simulink model "ts_b02f_log"  (R2024b)
settings: Solver=FixedStepDiscrete  StartTime=0.0  StopTime=10  FixedStep=Ts  RelTol=1e-4
PreLoadFcn:
  | Ts=50e-6;
undefined symbols (not defined in the file): D1, Delta, DiscIntNeverNeededParam
libraries: simulink x22, spsSecondOrderFilterLib x14, spsThreePhaseVIMeasurementLib x7, spsabctodq0Lib x6, spsThreePhaseSeriesRLCLoadLib x5, spsPowerPLLDrivenPositiveSequenceLib x4, spsStairGeneratorLib x4, spsThreePhaseTransformerTwoWindingsLib x3, spsDCVoltageSourceLib x3, spsThreePhaseSeriesRLCBranchLib x3, spsPWMGeneratorPulseAveragingLib x3, spsTwoLevelConverterLib x3
(part 3 of 3)

== system ts_b02f_log/Inverter 2 300 kW/Control System/Current Regulator/PI regulator with anti-windup D ==
  note: Anti-windup mechanism: Method of conditionnal integration
      |
      | The integration is suspended if saturation occurs and the
      | control error is of the same sign as the control signal.
      |
      | [1] L.Rundqwist, "Anti-Reset Windup for PID Controllers," Ph.D. Thesis TRFT-1033,
      | Departement of Automatic Control, Lund Institute of Technology, Lund, Sweeden, 1991.
  Error : Inport  SampleTime=Ts
  Compare To Zero : simulink/Logic and Bit Operations/Compare To Zero  relop=>  OutDataTypeStr=uint8  ZeroCross=off
  Compare To Zero1 : simulink/Logic and Bit Operations/Compare To Zero  relop=<  OutDataTypeStr=uint8  ZeroCross=off
  Constant : Constant  Value=0
  Constant1 : Constant  Value=UpperLimit
  Constant3 : Constant  Value=LowerLimit
  Discrete-Time Integrator : DiscreteIntegrator  IntegratorMethod=Integration: Trapezoidal  InitialCondition=Init  SampleTime=Ts  LimitOutput=on  UpperSaturationLimit=UpperLimit  LowerSaturationLimit=LowerLimit  ShowStatePort=on  ICPrevOutput=DiscIntNeverNeededParam  ICPrevScaledInput=DiscIntNeverNeededParam
  Kp4 : Gain  Gain=Kp  SaturateOnIntegerOverflow=on  SampleTime=Ts  OutDataTypeStr=Inherit: Same as input  ParamDataTypeStr=Inherit: Same as input
  Kp5 : Gain  Gain=Ki  SaturateOnIntegerOverflow=on  SampleTime=Ts  OutDataTypeStr=Inherit: Same as input  ParamDataTypeStr=Inherit: Same as input
  Logical Operator : Logic  AllPortsSameDT=off  OutDataTypeStr=boolean
  Logical Operator1 : Logic  AllPortsSameDT=off  OutDataTypeStr=boolean
  Logical Operator2 : Logic  Operator=OR  AllPortsSameDT=off  OutDataTypeStr=boolean
  Relational Operator : RelationalOperator  OutDataTypeStr=boolean  InputSameDT=off
  Relational Operator1 : RelationalOperator  Operator=<=  OutDataTypeStr=boolean  InputSameDT=off
  Saturation2 : Saturate  UpperLimit=UpperLimit  LowerLimit=LowerLimit  SampleTime=Ts
  Sum1 : Sum  InputSameDT=on  SaturateOnIntegerOverflow=on  SampleTime=Ts  OutDataTypeStr=Inherit: Same as first input
  Sum6 : Sum  InputSameDT=on  SaturateOnIntegerOverflow=on  SampleTime=Ts  OutDataTypeStr=Inherit: Same as first input
  Switch : Switch  Criteria=u2 > Threshold  SaturateOnIntegerOverflow=off  InputSameDT=off
  Zero-Order Hold : ZeroOrderHold  SampleTime=Ts
  Out : Outport  SampleTime=Ts  InitialOutput=0  VectorParamsAs1DForOutWhenUnconnected=off
  wires:
  Constant/1 -> Switch/1
  Zero-Order Hold/1 -> Sum1/2, Sum6/1
  Discrete-Time Integrator/State -> Sum1/1
  Sum1/1 -> Relational Operator1/1, Relational Operator/1
  Logical Operator2/1 -> Switch/2
  Relational Operator/1 -> Logical Operator/1  "UpperLimit_is_Reached"
  Relational Operator1/1 -> Logical Operator1/1  "LowerLimit_Is_Reached"
  Constant1/1 -> Relational Operator/2
  Constant3/1 -> Relational Operator1/2
  Compare To Zero/1 -> Logical Operator/2  "Error_is_positive"
  Logical Operator/1 -> Logical Operator2/1
  Logical Operator1/1 -> Logical Operator2/2
  Compare To Zero1/1 -> Logical Operator1/2  "Error_is_negative"
  Error/1 -> Compare To Zero1/1, Compare To Zero/1, Kp4/1, Kp5/1
  Sum6/1 -> Saturation2/1
  Kp4/1 -> Zero-Order Hold/1
  Discrete-Time Integrator/1 -> Sum6/2
  Saturation2/1 -> Out/1
  Switch/1 -> Discrete-Time Integrator/1
  Kp5/1 -> Switch/3

== system ts_b02f_log/Inverter 2 300 kW/Control System/Voltage Regulators/PI regulator with anti-windup 1 ==
  note: Anti-windup mechanism: Method of conditionnal integration
      |
      | The integration is suspended if saturation occurs and the
      | control error is of the same sign as the control signal.
      |
      | [1] L.Rundqwist, "Anti-Reset Windup for PID Controllers," Ph.D. Thesis TRFT-1033,
      | Departement of Automatic Control, Lund Institute of Technology, Lund, Sweeden, 1991.
  Error : Inport  SampleTime=Ts
  Reset : Inport  Port=2  SampleTime=Ts
  Compare To Zero : simulink/Logic and Bit Operations/Compare To Zero  relop=>  OutDataTypeStr=uint8  ZeroCross=off
  Compare To Zero1 : simulink/Logic and Bit Operations/Compare To Zero  relop=<  OutDataTypeStr=uint8  ZeroCross=off
  Constant : Constant  Value=0
  Constant1 : Constant  Value=UpperLimit
  Constant3 : Constant  Value=LowerLimit
  Discrete-Time Integrator : DiscreteIntegrator  IntegratorMethod=Integration: Trapezoidal  ExternalReset=level  InitialCondition=Init  SampleTime=Ts  LimitOutput=on  UpperSaturationLimit=UpperLimit  LowerSaturationLimit=LowerLimit  ShowStatePort=on  ICPrevOutput=DiscIntNeverNeededParam  ICPrevScaledInput=DiscIntNeverNeededParam
  Kp4 : Gain  Gain=Kp  SaturateOnIntegerOverflow=on  SampleTime=Ts  OutDataTypeStr=Inherit: Same as input  ParamDataTypeStr=Inherit: Same as input
  Kp5 : Gain  Gain=Ki  SaturateOnIntegerOverflow=on  SampleTime=Ts  OutDataTypeStr=Inherit: Same as input  ParamDataTypeStr=Inherit: Same as input
  Logical Operator : Logic  AllPortsSameDT=off  OutDataTypeStr=boolean
  Logical Operator1 : Logic  AllPortsSameDT=off  OutDataTypeStr=boolean
  Logical Operator2 : Logic  Operator=OR  AllPortsSameDT=off  OutDataTypeStr=boolean
  Relational Operator : RelationalOperator  OutDataTypeStr=boolean  InputSameDT=off
  Relational Operator1 : RelationalOperator  Operator=<=  OutDataTypeStr=boolean  InputSameDT=off
  Saturation2 : Saturate  UpperLimit=UpperLimit  LowerLimit=LowerLimit  SampleTime=Ts
  Sum1 : Sum  InputSameDT=on  SaturateOnIntegerOverflow=on  SampleTime=Ts  OutDataTypeStr=Inherit: Same as first input
  Sum6 : Sum  InputSameDT=on  SaturateOnIntegerOverflow=on  SampleTime=Ts  OutDataTypeStr=Inherit: Same as first input
  Switch : Switch  Criteria=u2 > Threshold  SaturateOnIntegerOverflow=off  InputSameDT=off
  Zero-Order Hold : ZeroOrderHold  SampleTime=Ts
  Out : Outport  SampleTime=Ts  InitialOutput=0  VectorParamsAs1DForOutWhenUnconnected=off
  wires:
  Kp5/1 -> Switch/3
  Switch/1 -> Discrete-Time Integrator/1
  Saturation2/1 -> Out/1
  Discrete-Time Integrator/1 -> Sum6/2
  Kp4/1 -> Zero-Order Hold/1
  Sum6/1 -> Saturation2/1
  Error/1 -> Kp5/1, Kp4/1, Compare To Zero/1, Compare To Zero1/1
  Compare To Zero1/1 -> Logical Operator1/2  "Error_is_negative"
  Logical Operator1/1 -> Logical Operator2/2
  Logical Operator/1 -> Logical Operator2/1
  Compare To Zero/1 -> Logical Operator/2  "Error_is_positive"
  Constant3/1 -> Relational Operator1/2
  Constant1/1 -> Relational Operator/2
  Relational Operator1/1 -> Logical Operator1/1  "LowerLimit_Is_Reached"
  Relational Operator/1 -> Logical Operator/1  "UpperLimit_is_Reached"
  Logical Operator2/1 -> Switch/2
  Sum1/1 -> Relational Operator/1, Relational Operator1/1
  Discrete-Time Integrator/State -> Sum1/1
  Zero-Order Hold/1 -> Sum6/1, Sum1/2
  Constant/1 -> Switch/1
  Reset/1 -> Discrete-Time Integrator/2

== system ts_b02f_log/Inverter 2 300 kW/Control System/Voltage Regulators/PI regulator with anti-windup 2 ==
  note: Anti-windup mechanism: Method of conditionnal integration
      |
      | The integration is suspended if saturation occurs and the
      | control error is of the same sign as the control signal.
      |
      | [1] L.Rundqwist, "Anti-Reset Windup for PID Controllers," Ph.D. Thesis TRFT-1033,
      | Departement of Automatic Control, Lund Institute of Technology, Lund, Sweeden, 1991.
  Error : Inport  SampleTime=Ts
  Reset : Inport  Port=2  SampleTime=Ts
  Compare To Zero : simulink/Logic and Bit Operations/Compare To Zero  relop=>  OutDataTypeStr=uint8  ZeroCross=off
  Compare To Zero1 : simulink/Logic and Bit Operations/Compare To Zero  relop=<  OutDataTypeStr=uint8  ZeroCross=off
  Constant : Constant  Value=0
  Constant1 : Constant  Value=UpperLimit
  Constant3 : Constant  Value=LowerLimit
  Discrete-Time Integrator : DiscreteIntegrator  IntegratorMethod=Integration: Trapezoidal  ExternalReset=level  InitialCondition=Init  SampleTime=Ts  LimitOutput=on  UpperSaturationLimit=UpperLimit  LowerSaturationLimit=LowerLimit  ShowStatePort=on  ICPrevOutput=DiscIntNeverNeededParam  ICPrevScaledInput=DiscIntNeverNeededParam
  Kp4 : Gain  Gain=Kp  SaturateOnIntegerOverflow=on  SampleTime=Ts  OutDataTypeStr=Inherit: Same as input  ParamDataTypeStr=Inherit: Same as input
  Kp5 : Gain  Gain=Ki  SaturateOnIntegerOverflow=on  SampleTime=Ts  OutDataTypeStr=Inherit: Same as input  ParamDataTypeStr=Inherit: Same as input
  Logical Operator : Logic  AllPortsSameDT=off  OutDataTypeStr=boolean
  Logical Operator1 : Logic  AllPortsSameDT=off  OutDataTypeStr=boolean
  Logical Operator2 : Logic  Operator=OR  AllPortsSameDT=off  OutDataTypeStr=boolean
  Relational Operator : RelationalOperator  OutDataTypeStr=boolean  InputSameDT=off
  Relational Operator1 : RelationalOperator  Operator=<=  OutDataTypeStr=boolean  InputSameDT=off
  Saturation2 : Saturate  UpperLimit=UpperLimit  LowerLimit=LowerLimit  SampleTime=Ts
  Sum1 : Sum  InputSameDT=on  SaturateOnIntegerOverflow=on  SampleTime=Ts  OutDataTypeStr=Inherit: Same as first input
  Sum6 : Sum  InputSameDT=on  SaturateOnIntegerOverflow=on  SampleTime=Ts  OutDataTypeStr=Inherit: Same as first input
  Switch : Switch  Criteria=u2 > Threshold  SaturateOnIntegerOverflow=off  InputSameDT=off
  Zero-Order Hold : ZeroOrderHold  SampleTime=Ts
  Out : Outport  SampleTime=Ts  InitialOutput=0  VectorParamsAs1DForOutWhenUnconnected=off
  wires:
  Kp5/1 -> Switch/3
  Switch/1 -> Discrete-Time Integrator/1
  Saturation2/1 -> Out/1
  Discrete-Time Integrator/1 -> Sum6/2
  Kp4/1 -> Zero-Order Hold/1
  Sum6/1 -> Saturation2/1
  Error/1 -> Kp5/1, Kp4/1, Compare To Zero/1, Compare To Zero1/1
  Compare To Zero1/1 -> Logical Operator1/2  "Error_is_negative"
  Logical Operator1/1 -> Logical Operator2/2
  Logical Operator/1 -> Logical Operator2/1
  Compare To Zero/1 -> Logical Operator/2  "Error_is_positive"
  Constant3/1 -> Relational Operator1/2
  Constant1/1 -> Relational Operator/2
  Relational Operator1/1 -> Logical Operator1/1  "LowerLimit_Is_Reached"
  Relational Operator/1 -> Logical Operator/1  "UpperLimit_is_Reached"
  Logical Operator2/1 -> Switch/2
  Sum1/1 -> Relational Operator/1, Relational Operator1/1
  Discrete-Time Integrator/State -> Sum1/1
  Zero-Order Hold/1 -> Sum6/1, Sum1/2
  Constant/1 -> Switch/1
  Reset/1 -> Discrete-Time Integrator/2

== system ts_b02f_log/Inverter 3 200 kW/Control System/Current Regulator/PI regulator with anti-windup D ==
  note: Anti-windup mechanism: Method of conditionnal integration
      |
      | The integration is suspended if saturation occurs and the
      | control error is of the same sign as the control signal.
      |
      | [1] L.Rundqwist, "Anti-Reset Windup for PID Controllers," Ph.D. Thesis TRFT-1033,
      | Departement of Automatic Control, Lund Institute of Technology, Lund, Sweeden, 1991.
  Error : Inport  SampleTime=Ts
  Compare To Zero : simulink/Logic and Bit Operations/Compare To Zero  relop=>  OutDataTypeStr=uint8  ZeroCross=off
  Compare To Zero1 : simulink/Logic and Bit Operations/Compare To Zero  relop=<  OutDataTypeStr=uint8  ZeroCross=off
  Constant : Constant  Value=0
  Constant1 : Constant  Value=UpperLimit
  Constant3 : Constant  Value=LowerLimit
  Discrete-Time Integrator : DiscreteIntegrator  IntegratorMethod=Integration: Trapezoidal  InitialCondition=Init  SampleTime=Ts  LimitOutput=on  UpperSaturationLimit=UpperLimit  LowerSaturationLimit=LowerLimit  ShowStatePort=on  ICPrevOutput=DiscIntNeverNeededParam  ICPrevScaledInput=DiscIntNeverNeededParam
  Kp4 : Gain  Gain=Kp  SaturateOnIntegerOverflow=on  SampleTime=Ts  OutDataTypeStr=Inherit: Same as input  ParamDataTypeStr=Inherit: Same as input
  Kp5 : Gain  Gain=Ki  SaturateOnIntegerOverflow=on  SampleTime=Ts  OutDataTypeStr=Inherit: Same as input  ParamDataTypeStr=Inherit: Same as input
  Logical Operator : Logic  AllPortsSameDT=off  OutDataTypeStr=boolean
  Logical Operator1 : Logic  AllPortsSameDT=off  OutDataTypeStr=boolean
  Logical Operator2 : Logic  Operator=OR  AllPortsSameDT=off  OutDataTypeStr=boolean
  Relational Operator : RelationalOperator  OutDataTypeStr=boolean  InputSameDT=off
  Relational Operator1 : RelationalOperator  Operator=<=  OutDataTypeStr=boolean  InputSameDT=off
  Saturation2 : Saturate  UpperLimit=UpperLimit  LowerLimit=LowerLimit  SampleTime=Ts
  Sum1 : Sum  InputSameDT=on  SaturateOnIntegerOverflow=on  SampleTime=Ts  OutDataTypeStr=Inherit: Same as first input
  Sum6 : Sum  InputSameDT=on  SaturateOnIntegerOverflow=on  SampleTime=Ts  OutDataTypeStr=Inherit: Same as first input
  Switch : Switch  Criteria=u2 > Threshold  SaturateOnIntegerOverflow=off  InputSameDT=off
  Zero-Order Hold : ZeroOrderHold  SampleTime=Ts
  Out : Outport  SampleTime=Ts  InitialOutput=0  VectorParamsAs1DForOutWhenUnconnected=off
  wires:
  Constant/1 -> Switch/1
  Zero-Order Hold/1 -> Sum1/2, Sum6/1
  Discrete-Time Integrator/State -> Sum1/1
  Sum1/1 -> Relational Operator1/1, Relational Operator/1
  Logical Operator2/1 -> Switch/2
  Relational Operator/1 -> Logical Operator/1  "UpperLimit_is_Reached"
  Relational Operator1/1 -> Logical Operator1/1  "LowerLimit_Is_Reached"
  Constant1/1 -> Relational Operator/2
  Constant3/1 -> Relational Operator1/2
  Compare To Zero/1 -> Logical Operator/2  "Error_is_positive"
  Logical Operator/1 -> Logical Operator2/1
  Logical Operator1/1 -> Logical Operator2/2
  Compare To Zero1/1 -> Logical Operator1/2  "Error_is_negative"
  Error/1 -> Compare To Zero1/1, Compare To Zero/1, Kp4/1, Kp5/1
  Sum6/1 -> Saturation2/1
  Kp4/1 -> Zero-Order Hold/1
  Discrete-Time Integrator/1 -> Sum6/2
  Saturation2/1 -> Out/1
  Switch/1 -> Discrete-Time Integrator/1
  Kp5/1 -> Switch/3

== system ts_b02f_log/Inverter 3 200 kW/Control System/Voltage Regulators/PI regulator with anti-windup 1 ==
  note: Anti-windup mechanism: Method of conditionnal integration
      |
      | The integration is suspended if saturation occurs and the
      | control error is of the same sign as the control signal.
      |
      | [1] L.Rundqwist, "Anti-Reset Windup for PID Controllers," Ph.D. Thesis TRFT-1033,
      | Departement of Automatic Control, Lund Institute of Technology, Lund, Sweeden, 1991.
  Error : Inport  SampleTime=Ts
  Reset : Inport  Port=2  SampleTime=Ts
  Compare To Zero : simulink/Logic and Bit Operations/Compare To Zero  relop=>  OutDataTypeStr=uint8  ZeroCross=off
  Compare To Zero1 : simulink/Logic and Bit Operations/Compare To Zero  relop=<  OutDataTypeStr=uint8  ZeroCross=off
  Constant : Constant  Value=0
  Constant1 : Constant  Value=UpperLimit
  Constant3 : Constant  Value=LowerLimit
  Discrete-Time Integrator : DiscreteIntegrator  IntegratorMethod=Integration: Trapezoidal  ExternalReset=level  InitialCondition=Init  SampleTime=Ts  LimitOutput=on  UpperSaturationLimit=UpperLimit  LowerSaturationLimit=LowerLimit  ShowStatePort=on  ICPrevOutput=DiscIntNeverNeededParam  ICPrevScaledInput=DiscIntNeverNeededParam
  Kp4 : Gain  Gain=Kp  SaturateOnIntegerOverflow=on  SampleTime=Ts  OutDataTypeStr=Inherit: Same as input  ParamDataTypeStr=Inherit: Same as input
  Kp5 : Gain  Gain=Ki  SaturateOnIntegerOverflow=on  SampleTime=Ts  OutDataTypeStr=Inherit: Same as input  ParamDataTypeStr=Inherit: Same as input
  Logical Operator : Logic  AllPortsSameDT=off  OutDataTypeStr=boolean
  Logical Operator1 : Logic  AllPortsSameDT=off  OutDataTypeStr=boolean
  Logical Operator2 : Logic  Operator=OR  AllPortsSameDT=off  OutDataTypeStr=boolean
  Relational Operator : RelationalOperator  OutDataTypeStr=boolean  InputSameDT=off
  Relational Operator1 : RelationalOperator  Operator=<=  OutDataTypeStr=boolean  InputSameDT=off
  Saturation2 : Saturate  UpperLimit=UpperLimit  LowerLimit=LowerLimit  SampleTime=Ts
  Sum1 : Sum  InputSameDT=on  SaturateOnIntegerOverflow=on  SampleTime=Ts  OutDataTypeStr=Inherit: Same as first input
  Sum6 : Sum  InputSameDT=on  SaturateOnIntegerOverflow=on  SampleTime=Ts  OutDataTypeStr=Inherit: Same as first input
  Switch : Switch  Criteria=u2 > Threshold  SaturateOnIntegerOverflow=off  InputSameDT=off
  Zero-Order Hold : ZeroOrderHold  SampleTime=Ts
  Out : Outport  SampleTime=Ts  InitialOutput=0  VectorParamsAs1DForOutWhenUnconnected=off
  wires:
  Kp5/1 -> Switch/3
  Switch/1 -> Discrete-Time Integrator/1
  Saturation2/1 -> Out/1
  Discrete-Time Integrator/1 -> Sum6/2
  Kp4/1 -> Zero-Order Hold/1
  Sum6/1 -> Saturation2/1
  Error/1 -> Kp5/1, Kp4/1, Compare To Zero/1, Compare To Zero1/1
  Compare To Zero1/1 -> Logical Operator1/2  "Error_is_negative"
  Logical Operator1/1 -> Logical Operator2/2
  Logical Operator/1 -> Logical Operator2/1
  Compare To Zero/1 -> Logical Operator/2  "Error_is_positive"
  Constant3/1 -> Relational Operator1/2
  Constant1/1 -> Relational Operator/2
  Relational Operator1/1 -> Logical Operator1/1  "LowerLimit_Is_Reached"
  Relational Operator/1 -> Logical Operator/1  "UpperLimit_is_Reached"
  Logical Operator2/1 -> Switch/2
  Sum1/1 -> Relational Operator/1, Relational Operator1/1
  Discrete-Time Integrator/State -> Sum1/1
  Zero-Order Hold/1 -> Sum6/1, Sum1/2
  Constant/1 -> Switch/1
  Reset/1 -> Discrete-Time Integrator/2

== system ts_b02f_log/Inverter 3 200 kW/Control System/Voltage Regulators/PI regulator with anti-windup 2 ==
  note: Anti-windup mechanism: Method of conditionnal integration
      |
      | The integration is suspended if saturation occurs and the
      | control error is of the same sign as the control signal.
      |
      | [1] L.Rundqwist, "Anti-Reset Windup for PID Controllers," Ph.D. Thesis TRFT-1033,
      | Departement of Automatic Control, Lund Institute of Technology, Lund, Sweeden, 1991.
  Error : Inport  SampleTime=Ts
  Reset : Inport  Port=2  SampleTime=Ts
  Compare To Zero : simulink/Logic and Bit Operations/Compare To Zero  relop=>  OutDataTypeStr=uint8  ZeroCross=off
  Compare To Zero1 : simulink/Logic and Bit Operations/Compare To Zero  relop=<  OutDataTypeStr=uint8  ZeroCross=off
  Constant : Constant  Value=0
  Constant1 : Constant  Value=UpperLimit
  Constant3 : Constant  Value=LowerLimit
  Discrete-Time Integrator : DiscreteIntegrator  IntegratorMethod=Integration: Trapezoidal  ExternalReset=level  InitialCondition=Init  SampleTime=Ts  LimitOutput=on  UpperSaturationLimit=UpperLimit  LowerSaturationLimit=LowerLimit  ShowStatePort=on  ICPrevOutput=DiscIntNeverNeededParam  ICPrevScaledInput=DiscIntNeverNeededParam
  Kp4 : Gain  Gain=Kp  SaturateOnIntegerOverflow=on  SampleTime=Ts  OutDataTypeStr=Inherit: Same as input  ParamDataTypeStr=Inherit: Same as input
  Kp5 : Gain  Gain=Ki  SaturateOnIntegerOverflow=on  SampleTime=Ts  OutDataTypeStr=Inherit: Same as input  ParamDataTypeStr=Inherit: Same as input
  Logical Operator : Logic  AllPortsSameDT=off  OutDataTypeStr=boolean
  Logical Operator1 : Logic  AllPortsSameDT=off  OutDataTypeStr=boolean
  Logical Operator2 : Logic  Operator=OR  AllPortsSameDT=off  OutDataTypeStr=boolean
  Relational Operator : RelationalOperator  OutDataTypeStr=boolean  InputSameDT=off
  Relational Operator1 : RelationalOperator  Operator=<=  OutDataTypeStr=boolean  InputSameDT=off
  Saturation2 : Saturate  UpperLimit=UpperLimit  LowerLimit=LowerLimit  SampleTime=Ts
  Sum1 : Sum  InputSameDT=on  SaturateOnIntegerOverflow=on  SampleTime=Ts  OutDataTypeStr=Inherit: Same as first input
  Sum6 : Sum  InputSameDT=on  SaturateOnIntegerOverflow=on  SampleTime=Ts  OutDataTypeStr=Inherit: Same as first input
  Switch : Switch  Criteria=u2 > Threshold  SaturateOnIntegerOverflow=off  InputSameDT=off
  Zero-Order Hold : ZeroOrderHold  SampleTime=Ts
  Out : Outport  SampleTime=Ts  InitialOutput=0  VectorParamsAs1DForOutWhenUnconnected=off
  wires:
  Kp5/1 -> Switch/3
  Switch/1 -> Discrete-Time Integrator/1
  Saturation2/1 -> Out/1
  Discrete-Time Integrator/1 -> Sum6/2
  Kp4/1 -> Zero-Order Hold/1
  Sum6/1 -> Saturation2/1
  Error/1 -> Kp5/1, Kp4/1, Compare To Zero/1, Compare To Zero1/1
  Compare To Zero1/1 -> Logical Operator1/2  "Error_is_negative"
  Logical Operator1/1 -> Logical Operator2/2
  Logical Operator/1 -> Logical Operator2/1
  Compare To Zero/1 -> Logical Operator/2  "Error_is_positive"
  Constant3/1 -> Relational Operator1/2
  Constant1/1 -> Relational Operator/2
  Relational Operator1/1 -> Logical Operator1/1  "LowerLimit_Is_Reached"
  Relational Operator/1 -> Logical Operator/1  "UpperLimit_is_Reached"
  Logical Operator2/1 -> Switch/2
  Sum1/1 -> Relational Operator/1, Relational Operator1/1
  Discrete-Time Integrator/State -> Sum1/1
  Zero-Order Hold/1 -> Sum6/1, Sum1/2
  Constant/1 -> Switch/1
  Reset/1 -> Discrete-Time Integrator/2
